simulink model "inverter"  (R2025b)
settings: Solver=ode23t  StartTime=0.0  StopTime=0.3  MaxStep=1e-5  RelTol=1e-3
libraries: ee_lib x16, fl_lib x13, nesl_utility x12, eeTransforms x2, slpidlib x1, eePwmGeneratorTwoLevel x1
settings Model: Creator=himal  LastModifiedBy=himal

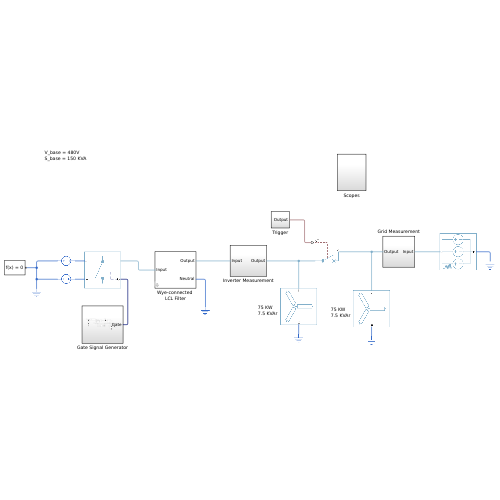
[thumbnail: Simulink's stored preview of the top-level diagram]
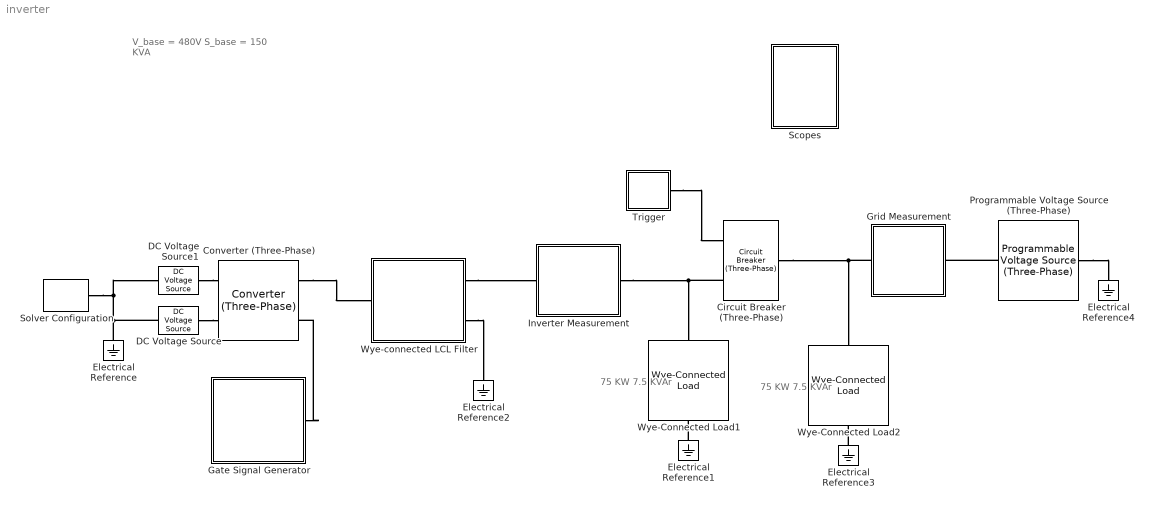
== system inverter ==
  note: V_base = 480V
      | S_base = 150 KVA
  note: 75 KW
      | 7.5 KVAr
  note: 75 KW
      | 7.5 KVAr
  Circuit Breaker (Three-Phase) : ee_lib/Switches & Breakers/Circuit Breaker (Three-Phase)  R_closed=0.001 Ohm  G_open=1e-6 1/Ohm  threshold=0.5 V  breaker_behavior=ee.enum.switches.breakerBehavior.zeroCrossingDisable
      settings: InternalSimscapePortConfiguration="{\"Bottom\":[],\"Left\":[{\"id\":\"vT\",\"label\":\"vT\",\"type\":\"input\"},{\"id\":\"N1\",\"label\":\"~1\",\"type\":\"foundation.electrical.three_phase\"}],\"Right\":[{\"id\":\"N2\",\"label\":\"~2\",\"type\":\"foundation.electrical.three_phase\"}],\"Top\":[]}"
  Converter (Three-Phase) : ee_lib/Semiconductors & Converters/Converters/Converter (Three-Phase)  port_option=ee.enum.threePhasePort.composite  fidelity_option=ee.enum.converters.fidelity.detailed  device_type=ee.enum.converters.switchingdevice.ideal  showThermalPort=false  K=0  Vth=0.5 V  Vgt=1 V  Vgt_off=-1 V  Ih=1 A  Vf=0.8 V  Ron=1e-3 Ohm  Rds=0.001 Ohm  Goff=2e-4 1/Ohm  Eon_scalar=22.86e-3 J  Eoff_scalar=17.14e-3 J  Eoff_natural_commutation=10e-3 J  Voff=300 V  Iout_scalar=600 A  onCurrentMeasDelay=0 s  useCurrentFromPreviousCycle=false  useVoltageFromPreviousCycle=false  diode_param=ee.enum.converters.protectiondiode.nodynamics  diode_Vf=0.8 V  diode_Ron=0.001 Ohm  diode_Goff=1e-5 1/Ohm  diode_C=50 nF  diode_iRM=-235 A  diode_iF=300 A  diode_idot=-50 A/us  diode_trr_param=ee.enum.converters.diodetrr.trr_factor  diode_trr_factor=3  diode_trr=15 us  diode_Qrr=1500 s*uA  diode_rec_loss_model=ee.enum.diode.reverseRecoveryModel.fixed  diode_ErecVal=0 J  diode_scaleWithIandV=false  diode_ErecMat=zeros(2, 3) J  diode_TjrecVec=[298.15, 398.15] K  diode_IfrecVec=[.1, 1, 10] A  diode_IrecVal=10 A  diode_VrecVal=10 V  diode_tFilter=1 / 1000 / 100 s  thermal_network_parameterization=ee.enum.thermalNetworkTopology.external  Rth=[.08, .5] K/W  Rth_Cauer=[.08, .1, .5] K/W  Rth_Foster=[.08, .14, .22, .16] K/W  thermal_mass_parameterization=ee.enum.thermalNetwork.timeconstant  thermal_mass=[.01, .5] J/K  thermal_mass_Cauer=[.01, .1, .5] J/K  thermal_mass_Foster=[.001, .005, .05, .5] J/K  thermal_time_constant=[.001, .2] s  thermal_time_constant_Cauer=[.001, .1, .2] s  thermal_time_constant_Foster=[7e-05, .0007, .01, .08] s  thermal_mass_initial_temperatures=[25, 25] degC  thermal_mass_initial_temperatures_Cauer=[25, 25, 25] degC  junction_thermal_mass=0.01 J/K  Tvec_initial_Foster=[25, 25, 25, 25] degC  snubber_type=ee.enum.converters.snubber.exclude  Cs=1e-7 F  Rs=0.1 Ohm  Vce_loss=[0, 150, 300] V
  DC Voltage Source : fl_lib/Electrical/Electrical Sources/DC Voltage Source  v0=500 V
  DC Voltage Source1 : fl_lib/Electrical/Electrical Sources/DC Voltage Source  v0=500 V
  Electrical Reference{,1..4} (5 alike) : fl_lib/Electrical/Electrical Elements/Electrical Reference
  Gate Signal Generator : Subsystem
  Grid Measurement : Subsystem
  Inverter Measurement : Subsystem
  Programmable Voltage Source (Three-Phase) : ee_lib/Sources/Programmable Voltage Source (Three-Phase)  magnitude_type=ee.enum.timechanging.constant  vline_rms=480 V  magn_ramp=1 V/s  magn_step=1 V  magn_modu_magn=1 V  magn_modu_freq=1 Hz  magn_t1=1 s  magn_t2=2 s  frequency_type=ee.enum.timechanging.constant  freq=50 Hz  freq_ramp=1 Hz/s  freq_step=1 Hz  freq_modu_magn=1 Hz  freq_modu_freq=1 Hz  freq_t1=1 s  freq_t2=2 s  phase_type=ee.enum.timechanging.constant  shift=0 deg  phase_ramp=1 deg/s  phase_step=1 deg  phase_modu_magn=1 deg  phase_modu_freq=1 Hz  phase_t1=1 s  phase_t2=2 s  impedance_option=1  SShortCircuit=1e6 A*V  XR=15  R=0.01 Ohm  L=3.97e-4 H  G_parasitic=1e-6 1/Ohm  harmonic_option=0  harmonic_orders=[5, 7, 11, 13]  harmonic_ratios=[.1, .1, .1, .1]  harmonic_shifts=[0, 0, 0, 0] deg  harmonic_sequences=[1, 1, 1, 1]  harmonic_t1=-inf s  harmonic_t2=inf s  I_specify=off  I_priority=None  I=[0, 0, 0] A  I_nominal_specify=off  I_nominal_value=1  I_nominal_unit=A  V_specify=off  V_priority=None  V=[0, 0, 0] V  V_nominal_specify=off  V_nominal_value=1  V_nominal_unit=V
      settings: InternalSimscapePortConfiguration="{\"Bottom\":[],\"Left\":[{\"id\":\"n\",\"label\":\"n\",\"type\":\"foundation.electrical.electrical\"}],\"Right\":[{\"id\":\"N\",\"label\":\"~\",\"type\":\"foundation.electrical.three_phase\"}],\"Top\":[]}"
  Scopes : Subsystem
  Solver Configuration : nesl_utility/Solver Configuration  PhysicalDomain=network_engine_domain  SubClassName=solver  LeftPortType=input  RightPortType=generic  Tones=[]  Harmonics=[]  SimulateNoise=off  Profile=off  UseLocalSampling=off  EnableSwitchedLinearOptims=on  FrequencyDomain=off  UseCCode=off  RelTol=0.001  AbsTol=0.001  MinStep=1e-09  ToWorkspace=off  RevertToSquareIcSolve=off  NumHomotopyIterations=100  PhasorMode=off  PhasorModeNumHarmonics=1  ConsistencySolver=NEWTON_XTOL_AFTER_FTOL  IndexReductionMethod=DerivativeReplacement  DoDC=off  ResidualTolerance=1e-09  ConsistencyTolSource=GLOBAL  ConsistencyAbsTol=0.001  ConsistencyRelTol=0.001  ConsistencyTolFactor=0.001  UseLocalSolver=off  LocalSolverChoice=NE_BACKWARD_EULER_ADVANCER  ResolveIndetEquations=on  FunctionEvalNumThread=1  LocalSolverSampleTime=0.001  DoFixedCost=off  MaxNonlinIter=3  MaxModeIter=2  ComputeImpulses=off  ImpulseIterations=2  LinearAlgebra=auto  LinearAlgebraNumThread=0  EquationFormulation=NE_TIME_EF  DelaysMemoryBudget=1024  AutomaticFiltering=on  FilteringTimeConstant=0.001  PartitionStorageMethod=AS_NEEDED  PartitionMemoryBudget=1024  PartitionMethod=ROBUST  MultibodyUseLocalSolver=off  MultibodyLocalSolverChoice=ODE1  MultibodyLocalSolverSampleTime=0.001
  Trigger : Subsystem
  Wye-Connected Load1 : ee_lib/Passive/RLC Assemblies/Wye-Connected Load  port_option=ee.enum.threePhasePort.composite  parameterization=ee.enum.rlc.parameterization.ratedpower  component_structure=ee.enum.rlc.structure.R  component_structure_PQ=ee.enum.rlc.structure.SeriesRL  R=1 Ohm  L=1e-3 H  C=1e-6 F  VRated=480/sqrt(3) V  FRated=50 Hz  P=75*1e3 W  Qpos=7500 A*V  Qneg=-3*1e3 A*V  R_parasitic=0 Ohm  G_parasitic=0 1/Ohm  R_parasitic_PQ=0 Ohm  G_parasitic_PQ=0 1/Ohm  Vmag0=0 V  Vang0=0 deg  Freq0=50 Hz  IL_specify=off  IL_priority=High  IL=[0, 0, 0] A  IL_nominal_specify=off  IL_nominal_value=1  IL_nominal_unit=A  VC_specify=off  VC_priority=High  VC=[0, 0, 0] V  VC_nominal_specify=off  VC_nominal_value=1  VC_nominal_unit=V
  Wye-Connected Load2 : ee_lib/Passive/RLC Assemblies/Wye-Connected Load  port_option=ee.enum.threePhasePort.composite  parameterization=ee.enum.rlc.parameterization.ratedpower  component_structure=ee.enum.rlc.structure.R  component_structure_PQ=ee.enum.rlc.structure.SeriesRL  R=1 Ohm  L=1e-3 H  C=1e-6 F  VRated=480/sqrt(3) V  FRated=50 Hz  P=75*1e3 W  Qpos=7500 A*V  Qneg=-3*1e3 A*V  R_parasitic=0 Ohm  G_parasitic=0 1/Ohm  R_parasitic_PQ=0 Ohm  G_parasitic_PQ=0 1/Ohm  Vmag0=0 V  Vang0=0 deg  Freq0=50 Hz  IL_specify=off  IL_priority=High  IL=[0, 0, 0] A  IL_nominal_specify=off  IL_nominal_value=1  IL_nominal_unit=A  VC_specify=off  VC_priority=High  VC=[0, 0, 0] V  VC_nominal_specify=off  VC_nominal_value=1  VC_nominal_unit=V
  Wye-connected LCL Filter : Subsystem  mask{L1=1e-3, C1=18*1e-4, L2=1e-3, Rd=0.5}
      mask prompts: L1 "Input Inductor"; C1 "Filter Capacitor"; L2 "Output Inductor"; Rd "Damping Resistor"
  connections:
  Electrical Reference1/LConn1 -- Wye-Connected Load1/RConn1
  Inverter Measurement/RConn1 -- Circuit Breaker (Three-Phase)/LConn2 -- Wye-Connected Load1/LConn1
  Electrical Reference3/LConn1 -- Wye-Connected Load2/RConn1
  Programmable Voltage Source (Three-Phase)/LConn1 -- Electrical Reference4/LConn1
  Trigger/RConn1 -- Circuit Breaker (Three-Phase)/LConn1
  Circuit Breaker (Three-Phase)/RConn1 -- Grid Measurement/RConn1 -- Wye-Connected Load2/LConn1
  Programmable Voltage Source (Three-Phase)/RConn1 -- Grid Measurement/LConn1
  Gate Signal Generator/RConn1 -- Converter (Three-Phase)/LConn1
  DC Voltage Source/RConn1 -- Solver Configuration/RConn1 -- DC Voltage Source1/LConn1 -- Electrical Reference/LConn1
  DC Voltage Source1/RConn1 -- Converter (Three-Phase)/RConn2
  DC Voltage Source/LConn1 -- Converter (Three-Phase)/RConn1
  Converter (Three-Phase)/LConn2 -- Wye-connected LCL Filter/LConn1
  Wye-connected LCL Filter/RConn1 -- Inverter Measurement/LConn1
  Wye-connected LCL Filter/RConn2 -- Electrical Reference2/LConn1

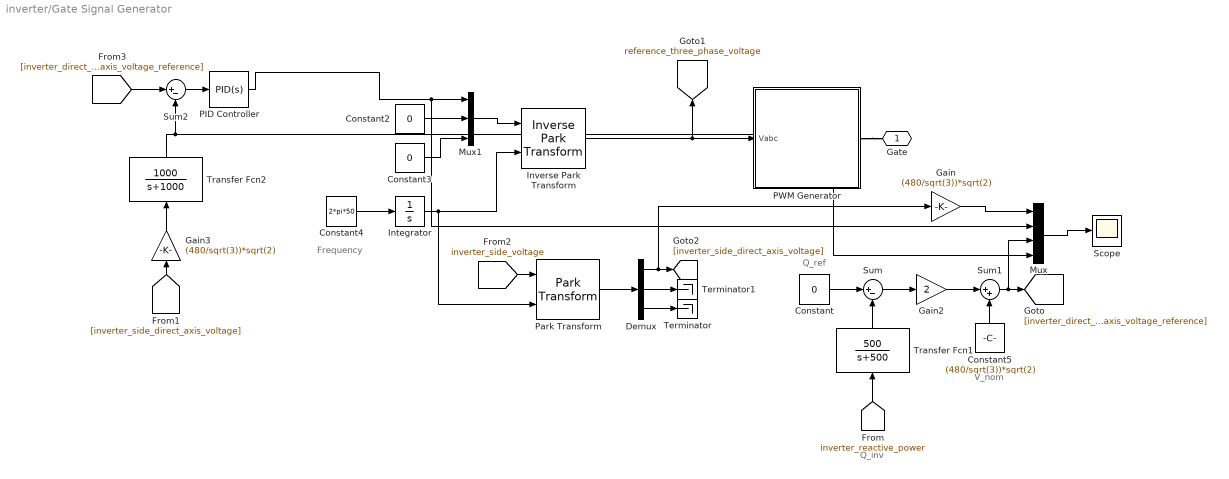
== system inverter/Gate Signal Generator ==
  note: Q_ref
  note: Q_inv
  note: V_nom
  note: Frequency
  Constant : Constant  Value=0
  Constant2 : Constant  Value=0
  Constant3 : Constant  Value=0
  Constant4 : Constant  Value=2*pi*50
  Constant5 : Constant  Value=(480/sqrt(3))*sqrt(2)
  Demux : Demux  Outputs=3
  Gain : Gain  Gain=(480/sqrt(3))*sqrt(2)
  Gain2 : Gain  Gain=2
  Gain3 : Gain  Gain=(480/sqrt(3))*sqrt(2)
  Integrator : Integrator  WrapState=on  WrappedStateUpperValue=2*pi  WrappedStateLowerValue=0
  Inverse Park Transform : eeTransforms/Inverse Park Transform  AxisAlignment=Q-axis  PowerInvariant=off
      settings: LibrarySourceBlock=|
      | ee_sl_lib/Mathematical
      | Transforms/Inverse
      | Park Transform
  Mux : Mux
  Mux1 : Mux  Inputs=3
  PID Controller : slpidlib/PID Controller  Controller=PID  Form=Parallel  TimeDomain=Continuous-time  UseExternalTs=off  SampleTime=-1  IntegratorMethod=Forward Euler  FilterMethod=Forward Euler  ControllerParametersSource=internal  P=1.0  I=350  UseKiTs=off  D=-0.2  UseExternalDerivativeSource=off  N=1  UseFilter=on  TunerSelectOption=Transfer Function Based (PID Tuner App)  InitialConditionSource=internal  InitialConditionForIntegrator=0  InitialConditionForFilter=0  DifferentiatorICPrevScaledInput=0  ExternalReset=none  TrackingMode=off  Kt=1  LimitOutput=off  SatLimitsSource=internal  UpperSaturationLimit=inf  LowerSaturationLimit=-inf  LinearizeAsGain=on  AntiWindupMode=none  Kb=1  LimitIntegrator=off  UpperIntegratorSaturationLimit=inf  LowerIntegratorSaturationLimit=-inf  POutMin=[]  POutMax=[]  IOutMin=[]  IOutMax=[]  DOutMin=[]  DOutMax=[]  NOutMin=[]  NOutMax=[]  SumOutMin=[]  SumOutMax=[]  SaturationOutMin=[]  SaturationOutMax=[]  PParamMin=[]  PParamMax=[]  IParamMin=[]  IParamMax=[]  DParamMin=[]  DParamMax=[]  NParamMin=[]  NParamMax=[]  KbParamMin=[]  KbParamMax=[]  KtParamMin=[]  KtParamMax=[]  KbOutMin=[]  KbOutMax=[]  KtOutMin=[]  KtOutMax=[]  IntegratorOutMin=[]  IntegratorOutMax=[]  FilterOutMin=[]  FilterOutMax=[]  SumI1OutMin=[]  SumI1OutMax=[]  SumI2OutMin=[]  SumI2OutMax=[]  SumI3OutMin=[]  SumI3OutMax=[]  SumI4OutMin=[]  SumI4OutMax=[]  SumDOutMin=[]  SumDOutMax=[]  DifferentiatorOutMin=[]  DifferentiatorOutMax=[]  FilterDiffOutCoefMin=[]  FilterDiffOutCoefMax=[]  ReciprocalOutMin=[]  ReciprocalOutMax=[]  SumDenOutMin=[]  SumDenOutMax=[]  SumNumOutMin=[]  SumNumOutMax=[]  DivideOutMin=[]  DivideOutMax=[]  UdiffTsProdOutMin=[]  UdiffTsProdOutMax=[]  NTsProdOutMin=[]  NTsProdOutMax=[]  UintegralTsProdOutMin=[]  UintegralTsProdOutMax=[]  UngainTsProdOutMin=[]  UngainTsProdOutMax=[]  ClampingZeroOutDataTypeStr=Inherit: Inherit via back propagation  ClampingZeroOutMin=[]  ClampingZeroOutMax=[]  FilterDenConstantOutDataTypeStr=Inherit: Inherit via back propagation  FilterDenConstantOutMin=[]  FilterDenConstantOutMax=[]  PCopyOutDataTypeStr=Inherit: Inherit via back propagation  PCopyOutMin=[]  PCopyOutMax=[]  NCopyOutDataTypeStr=Inherit: Inherit via back propagation  NCopyOutMin=[]  NCopyOutMax=[]  IntegratorContinuousStateAttributes=''  IntegratorStateMustResolveToSignalObject=off  IntegratorRTWStateStorageClass=Auto  FilterContinuousStateAttributes=''  FilterStateMustResolveToSignalObject=off  FilterRTWStateStorageClass=Auto  ParallelPVariant=InternalParameters  IdealPVariant=Disabled  IVariant=InternalParameters  DVariant=InternalParameters  IntegratorVariant=Continuous  SatVariant=Disabled  AWVariant=Passthrough  PCopyVariant=Disabled  TRVariant=Disabled  FdbkBlocksVariant=Forward  IdealPFdbkVariant=Disabled  SatFdbkVariant=Disabled  DerivativeFilterVariant=ContFilter  NVariant=InternalParameters  NCopyVariant=Disabled  FilterICVariant=InternalICsFilter  IntegratorICVariant=InternalICs  ExternalResetVariant=Disabled  TRSumVariant=Passthrough  SumFdbkVariant=Disabled  SumVariant=Sum_PID  TsampFilterVariant=InternalTs  TsampNgainVariant=Passthrough  TsampIntegralVariant=Disabled_SignalSpec  ExternalSaturationOutDataTypeStr=Inherit: Same as second input  DerivativeSourceVariant=ErrorSignal  PreIntVariant=InternalPreInt
  PWM Generator : Subsystem
  Park Transform : eeTransforms/Park Transform  AxisAlignment=Q-axis  PowerInvariant=off
      settings: LibrarySourceBlock=|
      | ee_sl_lib/Mathematical
      | Transforms/Park Transform
  Scope : Scope
      settings: ActiveDisplayYMinimum=-64.189678161126537  ActiveDisplayYMaximum=541.67390490064565  DataLoggingVariableName=ScopeData3
  Sum : Sum  Inputs=|+-
  Sum1 : Sum  Inputs=|++
  Sum2 : Sum  Inputs=|+-
  Terminator : Terminator
  Terminator1 : Terminator
  Transfer Fcn1 : TransferFcn  Numerator=[500]  Denominator=[1 500]
  Transfer Fcn2 : TransferFcn  Numerator=[1000]  Denominator=[1 1000]
  Gate : PMIOPort  Side=Right
  tag scope: reference_three_phase_voltage=global
  wires:
  Integrator/1 -> Park Transform/2, Inverse Park Transform/2
  Constant3/1 -> Mux1/3
  Constant4/1 -> Integrator/1
  Constant2/1 -> Mux1/2
  Mux1/1 -> Inverse Park Transform/1
  Inverse Park Transform/1 -> [reference_three_phase_voltage], PWM Generator/1(Vabc)
  Constant/1 -> Sum/1
  Constant5/1 -> Sum1/2
  Sum1/1 -> Mux/3, [inverter_direct_axis_voltage_reference]
  [inverter_side_voltage] -> Park Transform/1
  Park Transform/1 -> Demux/1
  Demux/3 -> Terminator/1
  Demux/2 -> Terminator1/1
  Demux/1 -> Gain/1, [inverter_side_direct_axis_voltage]
  Mux/1 -> Scope/1
  Gain/1 -> Mux/1
  Transfer Fcn1/1 -> Sum/2
  [inverter_reactive_power] -> Transfer Fcn1/1
  Sum/1 -> Gain2/1
  Gain2/1 -> Sum1/1
  [inverter_side_direct_axis_voltage] -> Gain3/1
  [inverter_direct_axis_voltage_reference] -> Sum2/1
  Sum2/1 -> PID Controller/1
  Gain3/1 -> Transfer Fcn2/1
  PID Controller/1 -> Mux/2, Mux1/1
  Transfer Fcn2/1 -> Mux/4, Sum2/2
  connections:
  PWM Generator/RConn1 -- Gate/RConn1

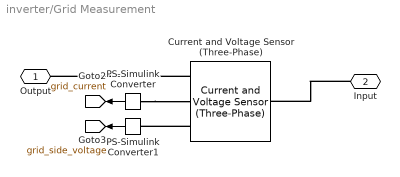
== system inverter/Grid Measurement ==
  Current and Voltage Sensor (Three-Phase) : ee_lib/Sensors & Transducers/Current and Voltage Sensor (Three-Phase)  vMeasurementType=ee.enum.vmeasurement.ll  outputUnit=ee.enum.unit.pu  SRated=150*1e3 A*V  VRated=480 V  I_specify=off  I_priority=None  I=[0, 0, 0] A  I_nominal_specify=off  I_nominal_value=1  I_nominal_unit=A  V_specify=off  V_priority=None  V=[0, 0, 0] V  V_nominal_specify=off  V_nominal_value=1  V_nominal_unit=V
      settings: InternalSimscapePortConfiguration="{\"Bottom\":[],\"Left\":[{\"id\":\"N1\",\"label\":\"~1\",\"type\":\"foundation.electrical.three_phase\"}],\"Right\":[{\"id\":\"V_output\",\"label\":\"V\",\"type\":\"output\"},{\"id\":\"I_output\",\"label\":\"I\",\"type\":\"output\"},{\"id\":\"N2\",\"label\":\"~2\",\"type\":\"foundation.electrical.three_phase\"}],\"Top\":[]}"
  PS-Simulink Converter : nesl_utility/PS-Simulink Converter  PhysicalDomain=network_engine_domain  SubClassName=ps_output  LeftPortType=input  RightPortType=output  PseudoPeriodic=off  Frequencies=[]  VectorFormat=inherit  Unit=inherit  AffineConversion=off
  PS-Simulink Converter1 : nesl_utility/PS-Simulink Converter  PhysicalDomain=network_engine_domain  SubClassName=ps_output  LeftPortType=input  RightPortType=output  PseudoPeriodic=off  Frequencies=[]  VectorFormat=inherit  Unit=inherit  AffineConversion=off
  Output : PMIOPort  Side=Right
  Input : PMIOPort  Port=2  Side=Left
  tag scope: grid_current=global, grid_side_voltage=global
  wires:
  PS-Simulink Converter1/1 -> [grid_side_voltage]
  PS-Simulink Converter/1 -> [grid_current]
  connections:
  PS-Simulink Converter/LConn1 -- Current and Voltage Sensor (Three-Phase)/RConn2
  Current and Voltage Sensor (Three-Phase)/RConn1 -- PS-Simulink Converter1/LConn1
  Current and Voltage Sensor (Three-Phase)/RConn3 -- Output/RConn1
  Input/RConn1 -- Current and Voltage Sensor (Three-Phase)/LConn1

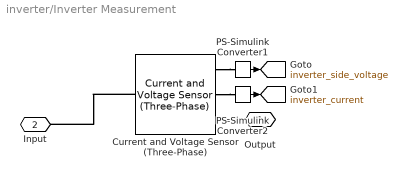
== system inverter/Inverter Measurement ==
  Current and Voltage Sensor (Three-Phase) : ee_lib/Sensors & Transducers/Current and Voltage Sensor (Three-Phase)  vMeasurementType=ee.enum.vmeasurement.ll  outputUnit=ee.enum.unit.pu  SRated=150*1e3 A*V  VRated=480 V  I_specify=off  I_priority=None  I=[0, 0, 0] A  I_nominal_specify=off  I_nominal_value=1  I_nominal_unit=A  V_specify=off  V_priority=None  V=[0, 0, 0] V  V_nominal_specify=off  V_nominal_value=1  V_nominal_unit=V
      settings: InternalSimscapePortConfiguration="{\"Bottom\":[],\"Left\":[{\"id\":\"N1\",\"label\":\"~1\",\"type\":\"foundation.electrical.three_phase\"}],\"Right\":[{\"id\":\"V_output\",\"label\":\"V\",\"type\":\"output\"},{\"id\":\"I_output\",\"label\":\"I\",\"type\":\"output\"},{\"id\":\"N2\",\"label\":\"~2\",\"type\":\"foundation.electrical.three_phase\"}],\"Top\":[]}"
  PS-Simulink Converter1 : nesl_utility/PS-Simulink Converter  PhysicalDomain=network_engine_domain  SubClassName=ps_output  LeftPortType=input  RightPortType=output  PseudoPeriodic=off  Frequencies=[]  VectorFormat=inherit  Unit=inherit  AffineConversion=off
  PS-Simulink Converter2 : nesl_utility/PS-Simulink Converter  PhysicalDomain=network_engine_domain  SubClassName=ps_output  LeftPortType=input  RightPortType=output  PseudoPeriodic=off  Frequencies=[]  VectorFormat=inherit  Unit=inherit  AffineConversion=off
  Output : PMIOPort  Side=Right
  Input : PMIOPort  Port=2  Side=Left
  tag scope: inverter_current=global, inverter_side_voltage=global
  wires:
  PS-Simulink Converter1/1 -> [inverter_side_voltage]
  PS-Simulink Converter2/1 -> [inverter_current]
  connections:
  Current and Voltage Sensor (Three-Phase)/LConn1 -- Input/RConn1
  Current and Voltage Sensor (Three-Phase)/RConn3 -- Output/RConn1
  Current and Voltage Sensor (Three-Phase)/RConn1 -- PS-Simulink Converter1/LConn1
  Current and Voltage Sensor (Three-Phase)/RConn2 -- PS-Simulink Converter2/LConn1

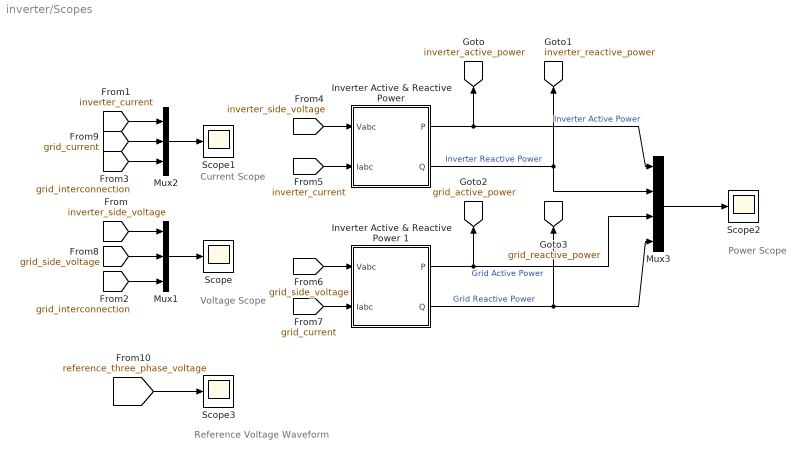
== system inverter/Scopes ==
  note: Reference
      | Voltage
      | Waveform
  note: Power
      | Scope
  note: Current
      | Scope
  note: Voltage
      | Scope
  "Inverter Active & Reactive Power " : Subsystem
  Inverter Active & Reactive Power 1 : Subsystem
  Mux1 : Mux  Inputs=3
  Mux2 : Mux  Inputs=3
  Mux3 : Mux
  Scope{,1..3} (4 alike) : Scope
      Scope settings: ActiveDisplayYMinimum=-1.2650918758334349  ActiveDisplayYMaximum=1.2710893448452796
      Scope1 settings: ActiveDisplayYMinimum=-2.8446347645381125  ActiveDisplayYMaximum=3.0929252622245289
      Scope2 settings: ActiveDisplayYMinimum=-1.2426998077724347  ActiveDisplayYMaximum=2.0955172958497728  DataLoggingVariableName=ScopeData2
      Scope3 settings: ActiveDisplayYMinimum=-1  ActiveDisplayYMaximum=1  DataLoggingVariableName=ScopeData4
  tag scope: grid_active_power=global, grid_reactive_power=global, inverter_active_power=global, inverter_reactive_power=global
  wires:
  [inverter_current] -> "Inverter Active & Reactive Power "/2(Iabc)
  Mux1/1 -> Scope/1
  [inverter_side_voltage] -> "Inverter Active & Reactive Power "/1(Vabc)
  [grid_side_voltage] -> Inverter Active & Reactive Power 1/1(Vabc)
  "Inverter Active & Reactive Power "/1(P) -> [inverter_active_power], Mux3/1  "Inverter Active Power"
  [grid_current] -> Inverter Active & Reactive Power 1/2(Iabc)
  Mux3/1 -> Scope2/1
  [inverter_side_voltage] -> Mux1/1
  "Inverter Active & Reactive Power "/2(Q) -> Mux3/2, [inverter_reactive_power]  "Inverter Reactive Power"
  Inverter Active & Reactive Power 1/1(P) -> [grid_active_power], Mux3/3  "Grid Active Power"
  Inverter Active & Reactive Power 1/2(Q) -> [grid_reactive_power], Mux3/4  "Grid Reactive Power"
  Mux2/1 -> Scope1/1
  [inverter_current] -> Mux2/1
  [grid_interconnection] -> Mux1/3
  [grid_side_voltage] -> Mux1/2
  [grid_interconnection] -> Mux2/3
  [grid_current] -> Mux2/2
  [reference_three_phase_voltage] -> Scope3/1

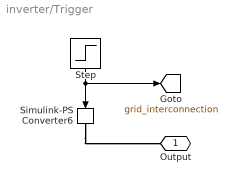
== system inverter/Trigger ==
  Simulink-PS Converter6 : nesl_utility/Simulink-PS Converter  PhysicalDomain=network_engine_domain  SubClassName=ps_input  LeftPortType=input  RightPortType=output  PseudoPeriodic=off  Frequencies=[]  NoiseDistribution=none  NoiseParameters=[]  Unit=1  AffineConversion=off  FilteringAndDerivatives=provide  SimscapeFilterOrder=1  InputFilterTimeConstant=0.001  UdotUserProvided=0
  Step : Step  Time=0.2  Before=1  After=0  SampleTime=0
  Output : PMIOPort  Side=Right
  tag scope: grid_interconnection=global
  wires:
  Step/1 -> [grid_interconnection], Simulink-PS Converter6/1
  connections:
  Simulink-PS Converter6/RConn1 -- Output/RConn1

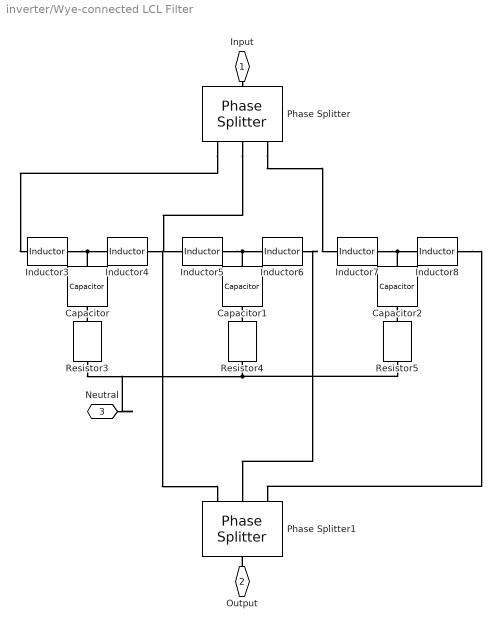
== system inverter/Wye-connected LCL Filter ==
  Capacitor : fl_lib/Electrical/Electrical Elements/Capacitor  c=C1 F  r=1e-6 Ohm  g=0 1/Ohm  i_specify=off  i_priority=None  i=0 A  i_nominal_specify=off  i_nominal_value=1  i_nominal_unit=A  v_specify=off  v_priority=None  v=0 V  v_nominal_specify=off  v_nominal_value=1  v_nominal_unit=V  vc_specify=off  vc_priority=High  vc=0 V  vc_nominal_specify=off  vc_nominal_value=1  vc_nominal_unit=V
  Capacitor1 : fl_lib/Electrical/Electrical Elements/Capacitor  c=C1 F  r=1e-6 Ohm  g=0 1/Ohm  i_specify=off  i_priority=None  i=0 A  i_nominal_specify=off  i_nominal_value=1  i_nominal_unit=A  v_specify=off  v_priority=None  v=0 V  v_nominal_specify=off  v_nominal_value=1  v_nominal_unit=V  vc_specify=off  vc_priority=High  vc=0 V  vc_nominal_specify=off  vc_nominal_value=1  vc_nominal_unit=V
  Capacitor2 : fl_lib/Electrical/Electrical Elements/Capacitor  c=C1 F  r=1e-6 Ohm  g=0 1/Ohm  i_specify=off  i_priority=None  i=0 A  i_nominal_specify=off  i_nominal_value=1  i_nominal_unit=A  v_specify=off  v_priority=None  v=0 V  v_nominal_specify=off  v_nominal_value=1  v_nominal_unit=V  vc_specify=off  vc_priority=High  vc=0 V  vc_nominal_specify=off  vc_nominal_value=1  vc_nominal_unit=V
  Inductor3 : ee_lib/Passive/Inductor  l=L1 H  enable_L_tol=ee.enum.toleranceApplication.none  L_tol=20  tol_distribution=ee.enum.toleranceDistribution.uniform  nSigma=4  r=0 Ohm  g=1e-9 1/Ohm  enable_operating_limits=ee.enum.enable.no  operating_limit_action=ee.enum.passive.reportOpLim.warn  max_working_current=1 A  power_rating=1 W  i_L_specify=off  i_L_priority=High  i_L=0 A  i_L_nominal_specify=off  i_L_nominal_value=1  i_L_nominal_unit=A
  Inductor4 : ee_lib/Passive/Inductor  l=L2 H  enable_L_tol=ee.enum.toleranceApplication.none  L_tol=20  tol_distribution=ee.enum.toleranceDistribution.uniform  nSigma=4  r=0 Ohm  g=1e-9 1/Ohm  enable_operating_limits=ee.enum.enable.no  operating_limit_action=ee.enum.passive.reportOpLim.warn  max_working_current=1 A  power_rating=1 W  i_L_specify=off  i_L_priority=High  i_L=0 A  i_L_nominal_specify=off  i_L_nominal_value=1  i_L_nominal_unit=A
  Inductor5 : ee_lib/Passive/Inductor  l=L1 H  enable_L_tol=ee.enum.toleranceApplication.none  L_tol=20  tol_distribution=ee.enum.toleranceDistribution.uniform  nSigma=4  r=0 Ohm  g=1e-9 1/Ohm  enable_operating_limits=ee.enum.enable.no  operating_limit_action=ee.enum.passive.reportOpLim.warn  max_working_current=1 A  power_rating=1 W  i_L_specify=off  i_L_priority=High  i_L=0 A  i_L_nominal_specify=off  i_L_nominal_value=1  i_L_nominal_unit=A
  Inductor6 : ee_lib/Passive/Inductor  l=L2 H  enable_L_tol=ee.enum.toleranceApplication.none  L_tol=20  tol_distribution=ee.enum.toleranceDistribution.uniform  nSigma=4  r=0 Ohm  g=1e-9 1/Ohm  enable_operating_limits=ee.enum.enable.no  operating_limit_action=ee.enum.passive.reportOpLim.warn  max_working_current=1 A  power_rating=1 W  i_L_specify=off  i_L_priority=High  i_L=0 A  i_L_nominal_specify=off  i_L_nominal_value=1  i_L_nominal_unit=A
  Inductor7 : ee_lib/Passive/Inductor  l=L1 H  enable_L_tol=ee.enum.toleranceApplication.none  L_tol=20  tol_distribution=ee.enum.toleranceDistribution.uniform  nSigma=4  r=0 Ohm  g=1e-9 1/Ohm  enable_operating_limits=ee.enum.enable.no  operating_limit_action=ee.enum.passive.reportOpLim.warn  max_working_current=1 A  power_rating=1 W  i_L_specify=off  i_L_priority=High  i_L=0 A  i_L_nominal_specify=off  i_L_nominal_value=1  i_L_nominal_unit=A
  Inductor8 : ee_lib/Passive/Inductor  l=L2 H  enable_L_tol=ee.enum.toleranceApplication.none  L_tol=20  tol_distribution=ee.enum.toleranceDistribution.uniform  nSigma=4  r=0 Ohm  g=1e-9 1/Ohm  enable_operating_limits=ee.enum.enable.no  operating_limit_action=ee.enum.passive.reportOpLim.warn  max_working_current=1 A  power_rating=1 W  i_L_specify=off  i_L_priority=High  i_L=0 A  i_L_nominal_specify=off  i_L_nominal_value=1  i_L_nominal_unit=A
  Phase Splitter : ee_lib/Connectors & References/Phase Splitter
  Phase Splitter1 : ee_lib/Connectors & References/Phase Splitter
  Resistor3 : fl_lib/Electrical/Electrical Elements/Resistor  R=Rd Ohm  i_specify=off  i_priority=None  i=0 A  i_nominal_specify=off  i_nominal_value=1  i_nominal_unit=A  v_specify=off  v_priority=None  v=0 V  v_nominal_specify=off  v_nominal_value=1  v_nominal_unit=V
  Resistor4 : fl_lib/Electrical/Electrical Elements/Resistor  R=Rd Ohm  i_specify=off  i_priority=None  i=0 A  i_nominal_specify=off  i_nominal_value=1  i_nominal_unit=A  v_specify=off  v_priority=None  v=0 V  v_nominal_specify=off  v_nominal_value=1  v_nominal_unit=V
  Resistor5 : fl_lib/Electrical/Electrical Elements/Resistor  R=Rd Ohm  i_specify=off  i_priority=None  i=0 A  i_nominal_specify=off  i_nominal_value=1  i_nominal_unit=A  v_specify=off  v_priority=None  v=0 V  v_nominal_specify=off  v_nominal_value=1  v_nominal_unit=V
  Input : PMIOPort  Side=Left
  Output : PMIOPort  Port=2  Side=Right
  Neutral : PMIOPort  Port=3  Side=Right
  connections:
  Resistor5/LConn1 -- Capacitor2/RConn1
  Inductor7/RConn1 -- Capacitor2/LConn1 -- Inductor8/LConn1
  Inductor3/RConn1 -- Capacitor/LConn1 -- Inductor4/LConn1
  Resistor5/RConn1 -- Resistor4/RConn1 -- Resistor3/RConn1 -- Neutral/RConn1
  Inductor6/RConn1 -- Phase Splitter1/RConn2
  Resistor3/LConn1 -- Capacitor/RConn1
  Inductor5/RConn1 -- Capacitor1/LConn1 -- Inductor6/LConn1
  Inductor8/RConn1 -- Phase Splitter1/RConn1
  Resistor4/LConn1 -- Capacitor1/RConn1
  Inductor4/RConn1 -- Phase Splitter1/RConn3
  Phase Splitter/RConn3 -- Inductor3/LConn1
  Phase Splitter/RConn2 -- Inductor5/LConn1
  Phase Splitter/RConn1 -- Inductor7/LConn1
  Input/RConn1 -- Phase Splitter/LConn1
  Output/RConn1 -- Phase Splitter1/LConn1

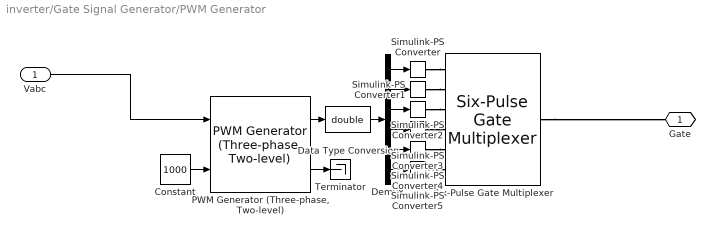
== system inverter/Gate Signal Generator/PWM Generator ==
  Vabc : Inport
  Constant : Constant  Value=1000
  Data Type Conversion : DataTypeConversion  OutDataTypeStr=double  SaturateOnIntegerOverflow=off  RndMeth=Floor
  Demux : Demux  Outputs=6
  "PWM Generator (Three-phase, Two-level)" : eePwmGeneratorTwoLevel/PWM Generator (Three-phase, Two-level)  PWMMode=Continuous PWM (CPWM)  CPWMMode=SVM: space vector modulation  DPWMMode=60 DPWM: 60 degree discontinuous PWM  fsw=1e4  Ts=5e-6
      settings: LibrarySourceBlock=|
      | ee_sl_lib/Pulse Width
      | Modulation/PWM Generator
      | (Three-phase, Two-level)
  Simulink-PS Converter{,1..5} (6 alike) : nesl_utility/Simulink-PS Converter  PhysicalDomain=network_engine_domain  SubClassName=ps_input  LeftPortType=input  RightPortType=output  PseudoPeriodic=off  Frequencies=[]  NoiseDistribution=none  NoiseParameters=[]  Unit=1  AffineConversion=off  FilteringAndDerivatives=provide  SimscapeFilterOrder=1  InputFilterTimeConstant=0.001  UdotUserProvided=0
  Six-Pulse Gate Multiplexer : ee_lib/Semiconductors & Converters/Converters/Six-Pulse Gate Multiplexer  port_option=ee.enum.controlport.ps
  Terminator : Terminator
  Gate : PMIOPort  Side=Right
  wires:
  Constant/1 -> "PWM Generator (Three-phase, Two-level)"/2
  "PWM Generator (Three-phase, Two-level)"/1 -> Data Type Conversion/1
  Demux/6 -> Simulink-PS Converter5/1
  Demux/1 -> Simulink-PS Converter/1
  "PWM Generator (Three-phase, Two-level)"/2 -> Terminator/1
  Demux/4 -> Simulink-PS Converter3/1
  Demux/2 -> Simulink-PS Converter1/1
  Demux/5 -> Simulink-PS Converter4/1
  Demux/3 -> Simulink-PS Converter2/1
  Data Type Conversion/1 -> Demux/1
  Vabc/1 -> "PWM Generator (Three-phase, Two-level)"/1
  connections:
  Simulink-PS Converter2/RConn1 -- Six-Pulse Gate Multiplexer/LConn3
  Six-Pulse Gate Multiplexer/RConn1 -- Gate/RConn1
  Simulink-PS Converter1/RConn1 -- Six-Pulse Gate Multiplexer/LConn2
  Simulink-PS Converter3/RConn1 -- Six-Pulse Gate Multiplexer/LConn4
  Simulink-PS Converter/RConn1 -- Six-Pulse Gate Multiplexer/LConn1
  Simulink-PS Converter5/RConn1 -- Six-Pulse Gate Multiplexer/LConn6
  Simulink-PS Converter4/RConn1 -- Six-Pulse Gate Multiplexer/LConn5

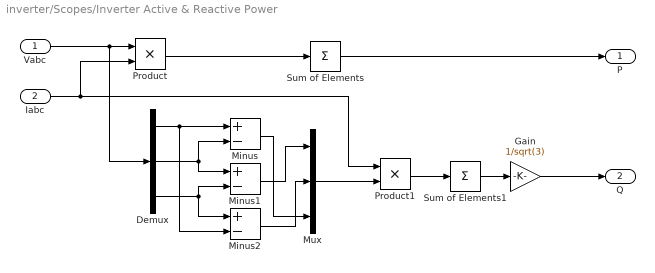
== system inverter/Scopes/Inverter Active & Reactive Power  ==
  Vabc : Inport
  Iabc : Inport  Port=2
  Demux : Demux  Outputs=3
  Gain : Gain  Gain=1/sqrt(3)
  Minus : Sum  Inputs=+-
  Minus1 : Sum  Inputs=+-
  Minus2 : Sum  Inputs=+-
  Mux : Mux  Inputs=3
  Product : Product
  Product1 : Product
  Sum of Elements : Sum  Inputs=+
  Sum of Elements1 : Sum  Inputs=+
  P : Outport  VectorParamsAs1DForOutWhenUnconnected=off
  Q : Outport  Port=2  VectorParamsAs1DForOutWhenUnconnected=off
  wires:
  Minus/1 -> Mux/3
  Minus2/1 -> Mux/2
  Minus1/1 -> Mux/1
  Gain/1 -> Q/1
  Sum of Elements1/1 -> Gain/1
  Product1/1 -> Sum of Elements1/1
  Mux/1 -> Product1/2
  Demux/3 -> Minus1/2, Minus2/1
  Demux/2 -> Minus/2, Minus1/1
  Demux/1 -> Minus/1, Minus2/2
  Sum of Elements/1 -> P/1
  Product/1 -> Sum of Elements/1
  Iabc/1 -> Product/2, Product1/1
  Vabc/1 -> Product/1, Demux/1

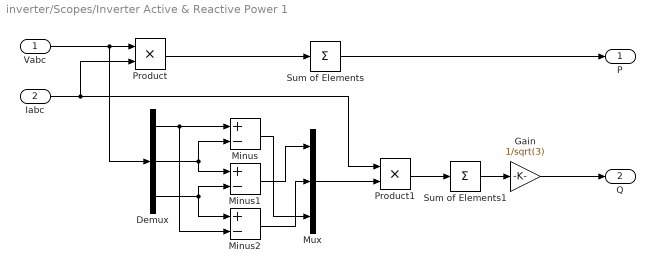
== system inverter/Scopes/Inverter Active & Reactive Power 1 ==
  Vabc : Inport
  Iabc : Inport  Port=2
  Demux : Demux  Outputs=3
  Gain : Gain  Gain=1/sqrt(3)
  Minus : Sum  Inputs=+-
  Minus1 : Sum  Inputs=+-
  Minus2 : Sum  Inputs=+-
  Mux : Mux  Inputs=3
  Product : Product
  Product1 : Product
  Sum of Elements : Sum  Inputs=+
  Sum of Elements1 : Sum  Inputs=+
  P : Outport  VectorParamsAs1DForOutWhenUnconnected=off
  Q : Outport  Port=2  VectorParamsAs1DForOutWhenUnconnected=off
  wires:
  Minus/1 -> Mux/3
  Minus2/1 -> Mux/2
  Minus1/1 -> Mux/1
  Gain/1 -> Q/1
  Sum of Elements1/1 -> Gain/1
  Product1/1 -> Sum of Elements1/1
  Mux/1 -> Product1/2
  Demux/3 -> Minus1/2, Minus2/1
  Demux/2 -> Minus/2, Minus1/1
  Demux/1 -> Minus/1, Minus2/2
  Sum of Elements/1 -> P/1
  Product/1 -> Sum of Elements/1
  Iabc/1 -> Product/2, Product1/1
  Vabc/1 -> Product/1, Demux/1
